simulink model "ELECTRIC_DRIVE"  (R2023a)
settings: Solver=ode1  StartTime=0.0  StopTime=tsim  FixedStep=CONTROL.Tm  RelTol=1e-3
undefined symbols (not defined in the file): CONTROL, MOTOR, myev, SENSOR, speed, tfalta, Tload, Vdc, VSC
libraries: simulink x9
(part 1 of 2)
settings Model: Creator=Usuario  LastModifiedBy=Usuario
settings DataIOCC: TimeSaveName=time  ReturnWorkspaceOutputsName=sim

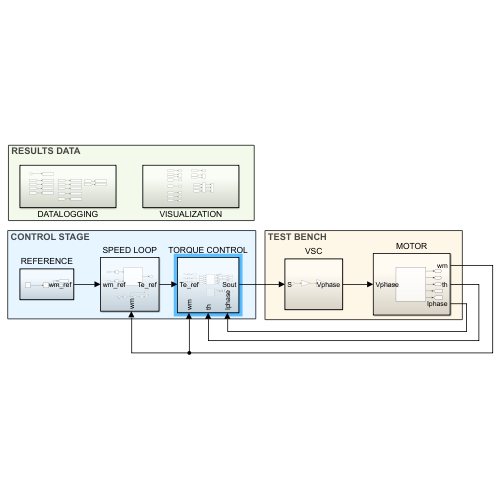
[thumbnail: Simulink's stored preview of the top-level diagram]
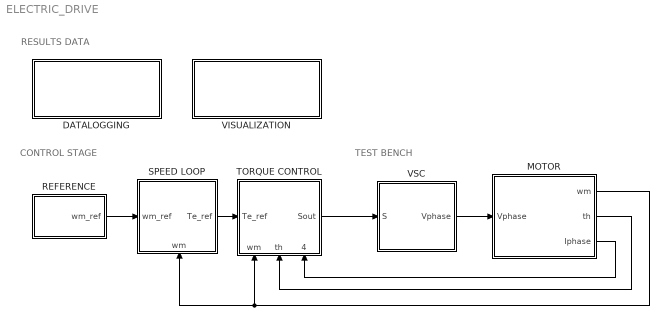
== system ELECTRIC_DRIVE ==
  note: RESULTS DATA
  note: TEST BENCH
  note: CONTROL STAGE
  DATALOGGING : Subsystem
  MOTOR : Subsystem
  REFERENCE : Subsystem
  SPEED LOOP : Subsystem
      settings: PortSchema="{\"entries\":[{\"content\":{\"sides\":[{\"content\":{\"connectorIds\":[\"In1\"]},\"type\":\"ConnectorPlacement.EquallySpacedRectSide\",\"uuid\":\"5121667f-51ba-4a0e-bd85-e87565fa1906\"},{\"content\":{\"connectorIds\":[\"Out1\"],\"side\":\"RIGHT\"},\"type\":\"ConnectorPlacement.EquallySpacedRectSide\",\"uuid\":\"7524861e-419c-49c4-ae4b-3a063630bebd\"},{\"content\":{\"side\":\"TOP\"},\"type\":\"ConnectorPlacement.EquallySpacedRectSide\",\"uuid\":\"8ed52486-91aa-4ff3-9364-bb7dbd5470e8\"},{\"content\":{\"connectorIds\":[\"In2\"],\"side\":\"BOTTOM\"},\"type\":\"ConnectorPlacement.EquallySpacedRectSide\",\"uuid\":\"0ee20b11-26ff-4e27-85a1-93f0e59c0d97\"}]},\"type\":\"ConnectorPlacement.EquallySpacedConnector\",\"uuid\":\"d6389f0f-3d9e-4163-a0bb-1bac6482b2ca\"}],\"packageUris\":[\"http://schema.mathworks.com/mf0/Connector/R2020b\"],\"version\":\"1.0\"}"
  TORQUE CONTROL : Subsystem
      settings: PortSchema="{\"entries\":[{\"content\":{\"sides\":[{\"content\":{\"connectorIds\":[\"In1\"]},\"type\":\"ConnectorPlacement.EquallySpacedRectSide\",\"uuid\":\"5121667f-51ba-4a0e-bd85-e87565fa1906\"},{\"content\":{\"connectorIds\":[\"Out1\"],\"side\":\"RIGHT\"},\"type\":\"ConnectorPlacement.EquallySpacedRectSide\",\"uuid\":\"7524861e-419c-49c4-ae4b-3a063630bebd\"},{\"content\":{\"side\":\"TOP\"},\"type\":\"ConnectorPlacement.EquallySpacedRectSide\",\"uuid\":\"8ed52486-91aa-4ff3-9364-bb7dbd5470e8\"},{\"content\":{\"connectorIds\":[\"In2\",\"In3\",\"In4\"],\"side\":\"BOTTOM\"},\"type\":\"ConnectorPlacement.EquallySpacedRectSide\",\"uuid\":\"eb3bd53b-f837-4c03-9b9f-2d851a494840\"}]},\"type\":\"ConnectorPlacement.EquallySpacedConnector\",\"uuid\":\"d6389f0f-3d9e-4163-a0bb-1bac6482b2ca\"}],\"packageUris\":[\"http://schema.mathworks.com/mf0/Connector/R2020b\"],\"version\":\"1.0\"}"
  VISUALIZATION : Subsystem
  VSC : Subsystem
  wires:
  REFERENCE/1(wm_ref) -> SPEED LOOP/1(wm_ref)
  SPEED LOOP/1(Te_ref) -> TORQUE CONTROL/1(Te_ref)
  TORQUE CONTROL/1(Sout) -> VSC/1(S)
  VSC/1(Vphase) -> MOTOR/1(Vphase)
  MOTOR/3(Iphase) -> TORQUE CONTROL/4(Iphase)
  MOTOR/1(wm) -> SPEED LOOP/2(wm), TORQUE CONTROL/2(wm)
  MOTOR/2(th) -> TORQUE CONTROL/3(th)

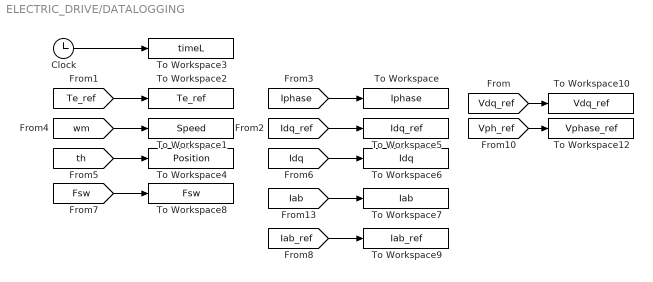
== system ELECTRIC_DRIVE/DATALOGGING ==
  Clock : Clock
  To Workspace : ToWorkspace  VariableName=Iphase  SampleTime=-1
      settings: Decimation=DEC
  To Workspace1 : ToWorkspace  VariableName=Speed  SampleTime=-1
      settings: Decimation=DEC
  To Workspace10 : ToWorkspace  VariableName=Vdq_ref  SampleTime=-1
      settings: Decimation=DEC
  To Workspace12 : ToWorkspace  VariableName=Vphase_ref  SampleTime=-1
      settings: Decimation=DEC
  To Workspace2 : ToWorkspace  VariableName=Te_ref  SampleTime=-1
      settings: Decimation=DEC
  To Workspace3 : ToWorkspace  VariableName=timeL  SampleTime=-1
      settings: Decimation=DEC
  To Workspace4 : ToWorkspace  VariableName=Position  SampleTime=-1
      settings: Decimation=DEC
  To Workspace5 : ToWorkspace  VariableName=Idq_ref  SampleTime=-1
      settings: Decimation=DEC
  To Workspace6 : ToWorkspace  VariableName=Idq  SampleTime=-1
      settings: Decimation=DEC
  To Workspace7 : ToWorkspace  VariableName=Iab  SampleTime=-1
      settings: Decimation=DEC
  To Workspace8 : ToWorkspace  VariableName=Fsw  SampleTime=-1
      settings: Decimation=DEC*100
  To Workspace9 : ToWorkspace  VariableName=Iab_ref  SampleTime=-1
      settings: Decimation=DEC
  wires:
  [Iphase] -> To Workspace/1
  [wm] -> To Workspace1/1
  Clock/1 -> To Workspace3/1
  [Te_ref] -> To Workspace2/1
  [th] -> To Workspace4/1
  [Idq_ref] -> To Workspace5/1
  [Idq] -> To Workspace6/1
  [Iab] -> To Workspace7/1
  [Fsw] -> To Workspace8/1
  [Iab_ref] -> To Workspace9/1
  [Vdq_ref] -> To Workspace10/1
  [Vph_ref] -> To Workspace12/1

== system ELECTRIC_DRIVE/MOTOR ==
  Vphase : Inport
  Variant Subsystem : Subsystem  Variant=on
  wm : Outport
  th : Outport  Port=2
  Iphase : Outport  Port=3
  tag scope: Iab=global, Idq=global
  wires:
  Vphase/1 -> Variant Subsystem/1(Vphase)
  Variant Subsystem/1(wm) -> wm/1
  Variant Subsystem/2(th) -> th/1
  Variant Subsystem/5(Iab) -> [Iab]
  Variant Subsystem/4(Idq) -> [Idq]
  Variant Subsystem/3(Iphase) -> Iphase/1

== system ELECTRIC_DRIVE/REFERENCE ==
  Ramp : simulink/Sources/Ramp  slope=14*speed*2*pi/60  start=0  InitialOutput=0
  Saturation : Saturate  UpperLimit=speed*2*pi/60  LowerLimit=0
  wm_ref : Outport
  tag scope: wm_ref=global
  wires:
  Ramp/1 -> Saturation/1
  Saturation/1 -> [wm_ref], wm_ref/1

== system ELECTRIC_DRIVE/SPEED LOOP ==
  wm_ref : Inport
  wm : Inport  Port=2
  Add : Sum  Commented=on
  Integrator : Integrator  Commented=on
  Ki : Gain  Commented=on  Gain=CONTROL.VEL.Ki
  Kp : Gain  Commented=on  Gain=CONTROL.VEL.Kp
  SPEED PI CONTROLLER : MATLAB Function  Description=OEW MPC VV 5PH  TreatAsAtomicUnit=on
  Sum : Sum  Commented=on  Inputs=|+-
  Transport Delay : TransportDelay  DelayTime=CONTROL.Ts - CONTROL.Tm
  Transport Delay1 : TransportDelay  DelayTime=CONTROL.Ts - CONTROL.Tm
  Te_ref : Outport
  wires:
  Sum/1 -> Kp/1
  Ki/1 -> Integrator/1
  Integrator/1 -> Add/2
  Kp/1 -> Add/1, Ki/1
  wm_ref/1 -> Transport Delay/1
  wm/1 -> Transport Delay1/1
  SPEED PI CONTROLLER/1(T_ref) -> Te_ref/1
  Transport Delay/1 -> SPEED PI CONTROLLER/1(wm_ref)
  Transport Delay1/1 -> SPEED PI CONTROLLER/2(wm)

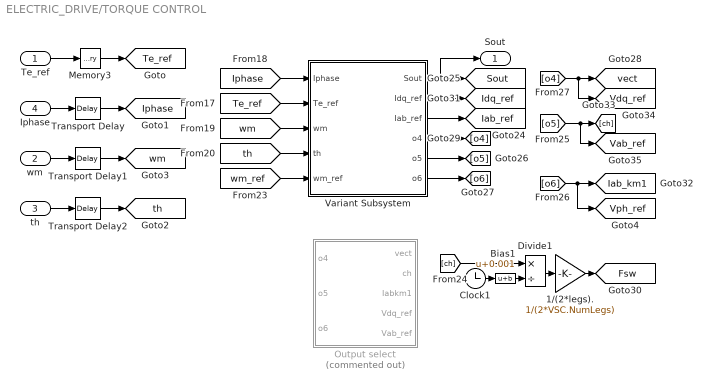
== system ELECTRIC_DRIVE/TORQUE CONTROL ==
  Te_ref : Inport
  wm : Inport  Port=2
  th : Inport  Port=3
  Iphase : Inport  Port=4
  1/(2*legs). : Gain  Gain=1/(2*VSC.NumLegs)
  Bias1 : Bias  Bias=0.001  SaturateOnIntegerOverflow=off
  Clock1 : Clock
  Divide1 : Product  Inputs=*/
  Memory3 : Memory
  Output select : MATLAB Function  Commented=on  TreatAsAtomicUnit=on
  Transport Delay : TransportDelay  DelayTime=CONTROL.Ts - CONTROL.Tm
  Transport Delay1 : TransportDelay  DelayTime=CONTROL.Ts - CONTROL.Tm
  Transport Delay2 : TransportDelay  DelayTime=CONTROL.Ts - CONTROL.Tm
  Variant Subsystem : Subsystem  Variant=on
  Sout : Outport
  tag scope: Fsw=global, Iab_km1=global, Iab_ref=global, Idq_ref=global, Iphase=global, Sout=global, Te_ref=global, Vab_ref=global, Vdq_ref=global, Vph_ref=global, th=global, vect=global, wm=global
  wires:
  Te_ref/1 -> Memory3/1
  Iphase/1 -> Transport Delay/1
  wm/1 -> Transport Delay1/1
  Transport Delay/1 -> [Iphase]
  Memory3/1 -> [Te_ref]
  th/1 -> Transport Delay2/1
  Transport Delay1/1 -> [wm]
  Transport Delay2/1 -> [th]
  [Iphase] -> Variant Subsystem/1(Iphase)
  [Te_ref] -> Variant Subsystem/2(Te_ref)
  [wm] -> Variant Subsystem/3(wm)
  [th] -> Variant Subsystem/4(th)
  [wm_ref] -> Variant Subsystem/5(wm_ref)
  Clock1/1 -> Bias1/1
  Bias1/1 -> Divide1/2
  1/(2*legs)./1 -> [Fsw]
  Divide1/1 -> 1/(2*legs)./1
  Variant Subsystem/1(Sout) -> Sout/1, [Sout]
  Variant Subsystem/4(o4) -> [o4]
  Variant Subsystem/2(Idq_ref) -> [Idq_ref]
  Variant Subsystem/3(Iab_ref) -> [Iab_ref]
  Variant Subsystem/6(o6) -> [o6]
  Variant Subsystem/5(o5) -> [o5]
  [ch] -> Divide1/1
  [o4] -> [Vdq_ref], [vect]
  [o5] -> [Vab_ref], [ch]
  [o6] -> [Vph_ref], [Iab_km1]

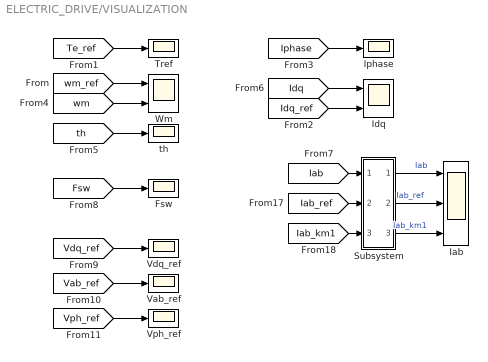
== system ELECTRIC_DRIVE/VISUALIZATION ==
  Fsw : Scope
  Iab : Scope  NumInputPorts=3
  Idq : Scope  NumInputPorts=2
  Iphase : Scope
  Subsystem : Subsystem
  Tref : Scope
  Vab_ref : Scope
  Vdq_ref : Scope
  Vph_ref : Scope
  Wm : Scope  NumInputPorts=2
  th : Scope
  wires:
  [th] -> th/1
  [Te_ref] -> Tref/1
  [wm] -> Wm/2
  [Iphase] -> Iphase/1
  [wm_ref] -> Wm/1
  [Iab] -> Subsystem/1(In1)
  [Iab_ref] -> Subsystem/2(In2)
  [Iab_km1] -> Subsystem/3(In3)
  Subsystem/1(Out1) -> Iab/1  "Iab"
  Subsystem/2(Out2) -> Iab/2  "Iab_ref"
  Subsystem/3(Out3) -> Iab/3  "Iab_km1"
  [Fsw] -> Fsw/1
  [Vdq_ref] -> Vdq_ref/1
  [Vab_ref] -> Vab_ref/1
  [Vph_ref] -> Vph_ref/1
  [Idq] -> Idq/1
  [Idq_ref] -> Idq/2

== system ELECTRIC_DRIVE/VSC ==
  S : Inport
  VSC Model : Gain  Gain=VSC.K  Multiplication=Matrix(K*u)
  Vdc : Gain  Gain=VSC.Vdc
  Vphase : Outport
  wires:
  S/1 -> Vdc/1
  VSC Model/1 -> Vphase/1
  Vdc/1 -> VSC Model/1

== system ELECTRIC_DRIVE/MOTOR/Variant Subsystem ==
  note: 1) Add Subsystem or Model blocks as valid variant choices.
      | 2) You cannot connect blocks at this level. At simulation, connectivity is automatically
      | determined, based on the active variant and port name matching.
  Vphase : Inport
  IM_5Ph : Subsystem  VariantControl=MOTOR.Index == 2
  IM_6Ph : Subsystem  VariantControl=MOTOR.Index == 6
  PMSM_5Ph : Subsystem  VariantControl=MOTOR.Index == 1
  PMSM_9Ph : Subsystem  VariantControl=MOTOR.Index == 3
  wm : Outport
  th : Outport  Port=2
  Iphase : Outport  Port=3
  Idq : Outport  Port=4
  Iab : Outport  Port=5

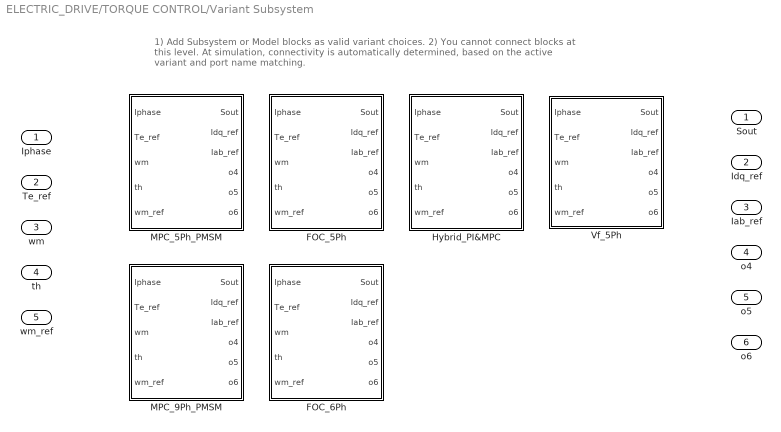
== system ELECTRIC_DRIVE/TORQUE CONTROL/Variant Subsystem ==
  note: 1) Add Subsystem or Model blocks as valid variant choices.
      | 2) You cannot connect blocks at this level. At simulation, connectivity is automatically
      | determined, based on the active variant and port name matching.
  Iphase : Inport
  Te_ref : Inport  Port=2
  wm : Inport  Port=3
  th : Inport  Port=4
  wm_ref : Inport  Port=5
  FOC_5Ph : Subsystem  VariantControl=CONTROL.Index == 52
  FOC_6Ph : Subsystem  VariantControl=CONTROL.Index == 52
  Hybrid_PI&MPC : Subsystem  VariantControl=CONTROL.Index == 53
  MPC_5Ph_PMSM : Subsystem  VariantControl=CONTROL.Index == 51
  MPC_9Ph_PMSM : Subsystem  VariantControl=CONTROL.Index == 91
  Vf_5Ph : Subsystem  VariantControl=CONTROL.Index == 55
  Sout : Outport
  Idq_ref : Outport  Port=2
  Iab_ref : Outport  Port=3
  o4 : Outport  Port=4
  o5 : Outport  Port=5
  o6 : Outport  Port=6

== system ELECTRIC_DRIVE/VISUALIZATION/Subsystem ==
  In1 : Inport
  In2 : Inport  Port=2
  In3 : Inport  Port=3
  Demux1 : Demux  Outputs=[2 3]
  Demux2 : Demux  Outputs=[2 3]
  Out1 : Outport
  Out2 : Outport  Port=2
  Out3 : Outport  Port=3
  wires:
  In1/1 -> Out1/1
  In2/1 -> Demux1/1
  In3/1 -> Demux2/1
  Demux2/1 -> Out3/1
  Demux1/1 -> Out2/1

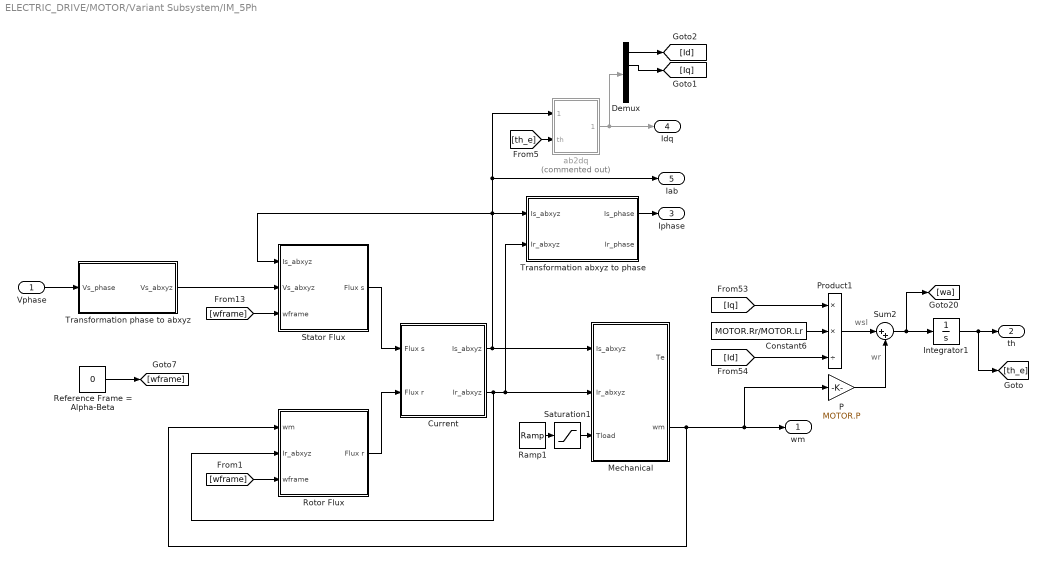
== system ELECTRIC_DRIVE/MOTOR/Variant Subsystem/IM_5Ph ==
  note: wr
  note: wsl
  Vphase : Inport
  Constant6 : Constant  Value=MOTOR.Rr/MOTOR.Lr
  Current : Subsystem
  Demux : Demux
  Integrator1 : Integrator
  Mechanical : Subsystem
  P : Gain  Gain=MOTOR.P
  Product1 : Product  Inputs=**/  RndMeth=Zero
  Ramp1 : simulink/Sources/Ramp  slope=40*Tload  start=0  InitialOutput=0
  Reference Frame = Alpha-Beta : Constant  Value=0
  Rotor Flux : Subsystem
  Saturation1 : Saturate  UpperLimit=Tload  LowerLimit=0
  "Stator Flux " : Subsystem
  Sum2 : Sum  Inputs=|++
  Transformation abxyz to phase : Subsystem
  Transformation phase to abxyz : Subsystem
  ab2dq : MATLAB Function  Commented=on  TreatAsAtomicUnit=on
  wm : Outport  VectorParamsAs1DForOutWhenUnconnected=off
  th : Outport  Port=2  VectorParamsAs1DForOutWhenUnconnected=off
  Iphase : Outport  Port=3  VectorParamsAs1DForOutWhenUnconnected=off
  Idq : Outport  Port=4  VectorParamsAs1DForOutWhenUnconnected=off
  Iab : Outport  Port=5  VectorParamsAs1DForOutWhenUnconnected=off
  wires:
  [wframe] -> "Stator Flux "/3(wframe)
  Transformation phase to abxyz/1(Vs_abxyz) -> "Stator Flux "/2(Vs_abxyz)
  Ramp1/1 -> Saturation1/1
  Vphase/1 -> Transformation phase to abxyz/1(Vs_phase)
  Current/2(Ir_abxyz) -> Rotor Flux/2(Ir_abxyz), Transformation abxyz to phase/2(Ir_abxyz), Mechanical/2(Ir_abxyz)
  Current/1(Is_abxyz) -> ab2dq/1(Vabxy), Iab/1, Transformation abxyz to phase/1(Is_abxyz), "Stator Flux "/1(Is_abxyz), Mechanical/1(Is_abxyz)
  "Stator Flux "/1(Flux s) -> Current/1(Flux s)
  Reference Frame = Alpha-Beta/1 -> [wframe]
  Rotor Flux/1(Flux r) -> Current/2(Flux r)
  [wframe] -> Rotor Flux/3(wframe)
  Saturation1/1 -> Mechanical/3(Tload)
  Transformation abxyz to phase/1(Is_phase) -> Iphase/1
  Integrator1/1 -> [th_e], th/1
  [th_e] -> ab2dq/2(th)
  ab2dq/1(Vdqxy) -> Demux/1, Idq/1
  P/1 -> Sum2/2
  Product1/1 -> Sum2/1
  [Id] -> Product1/3
  Mechanical/2(wm) -> P/1, wm/1, Rotor Flux/1(wm)
  Sum2/1 -> Integrator1/1, [wa]
  Constant6/1 -> Product1/2
  [Iq] -> Product1/1
  Demux/2 -> [Iq]
  Demux/1 -> [Id]

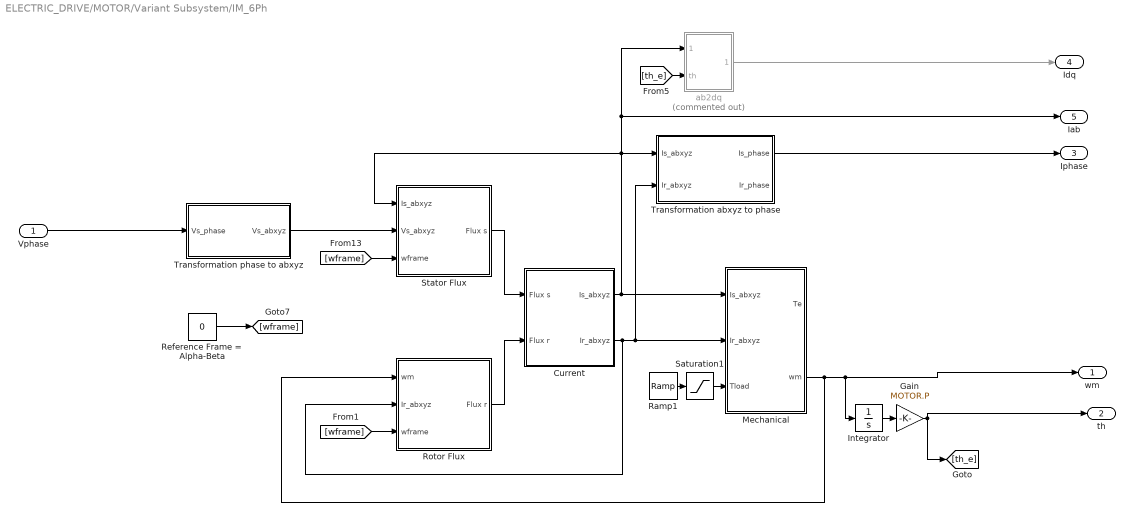
== system ELECTRIC_DRIVE/MOTOR/Variant Subsystem/IM_6Ph ==
  Vphase : Inport
  Current : Subsystem
  Gain : Gain  Gain=MOTOR.P
  Integrator : Integrator
  Mechanical : Subsystem
  Ramp1 : simulink/Sources/Ramp  slope=40*Tload  start=0  InitialOutput=0
  Reference Frame = Alpha-Beta : Constant  Value=0
  Rotor Flux : Subsystem
  Saturation1 : Saturate  UpperLimit=Tload  LowerLimit=0
  "Stator Flux " : Subsystem
  Transformation abxyz to phase : Subsystem
  Transformation phase to abxyz : Subsystem
  ab2dq : MATLAB Function  Commented=on  TreatAsAtomicUnit=on
  wm : Outport  VectorParamsAs1DForOutWhenUnconnected=off
  th : Outport  Port=2  VectorParamsAs1DForOutWhenUnconnected=off
  Iphase : Outport  Port=3  VectorParamsAs1DForOutWhenUnconnected=off
  Idq : Outport  Port=4  VectorParamsAs1DForOutWhenUnconnected=off
  Iab : Outport  Port=5  VectorParamsAs1DForOutWhenUnconnected=off
  wires:
  ab2dq/1(Vdqxy) -> Idq/1
  [th_e] -> ab2dq/2(th)
  Gain/1 -> th/1, [th_e]
  Integrator/1 -> Gain/1
  Transformation abxyz to phase/1(Is_phase) -> Iphase/1
  Saturation1/1 -> Mechanical/3(Tload)
  [wframe] -> Rotor Flux/3(wframe)
  Rotor Flux/1(Flux r) -> Current/2(Flux r)
  Mechanical/2(wm) -> Rotor Flux/1(wm), wm/1, Integrator/1
  Reference Frame = Alpha-Beta/1 -> [wframe]
  "Stator Flux "/1(Flux s) -> Current/1(Flux s)
  Current/1(Is_abxyz) -> Mechanical/1(Is_abxyz), "Stator Flux "/1(Is_abxyz), Transformation abxyz to phase/1(Is_abxyz), Iab/1, ab2dq/1(Vabxy)
  Current/2(Ir_abxyz) -> Mechanical/2(Ir_abxyz), Transformation abxyz to phase/2(Ir_abxyz), Rotor Flux/2(Ir_abxyz)
  Vphase/1 -> Transformation phase to abxyz/1(Vs_phase)
  Ramp1/1 -> Saturation1/1
  Transformation phase to abxyz/1(Vs_abxyz) -> "Stator Flux "/2(Vs_abxyz)
  [wframe] -> "Stator Flux "/3(wframe)

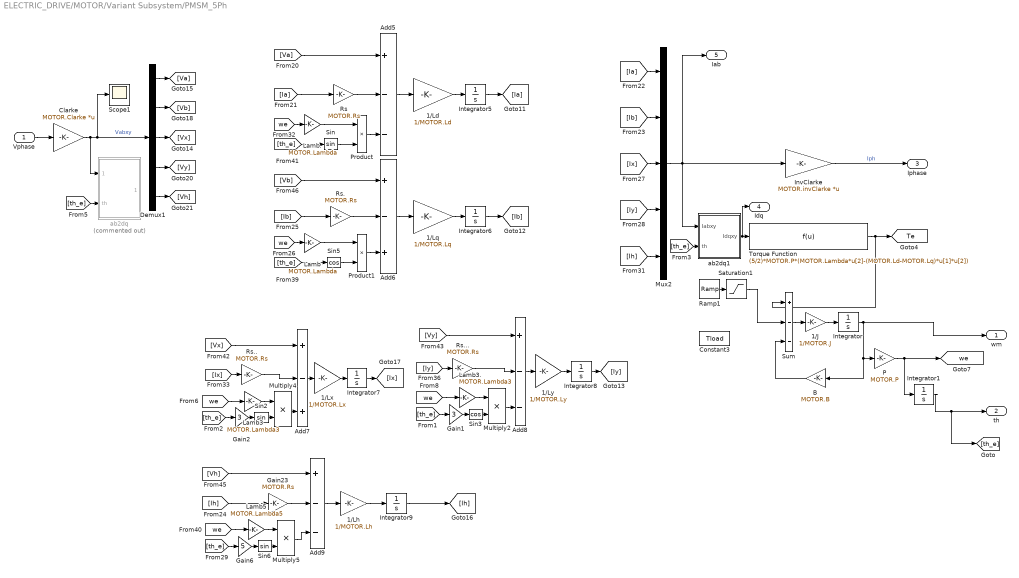
== system ELECTRIC_DRIVE/MOTOR/Variant Subsystem/PMSM_5Ph ==
  Vphase : Inport
  1/J : Gain  Gain=1/MOTOR.J
  1/Ld : Gain  Gain=1/MOTOR.Ld
  1/Lh : Gain  Gain=1/MOTOR.Lh
  1/Lq : Gain  Gain=1/MOTOR.Lq
  1/Lx : Gain  Gain=1/MOTOR.Lx
  1/Ly : Gain  Gain=1/MOTOR.Ly
  Add5 : Sum  Inputs=+--
  Add6 : Sum  Inputs=+-+
  Add7 : Sum  Inputs=+-+
  Add8 : Sum  Inputs=+--
  Add9 : Sum  Inputs=+--
  B : Gain  Gain=MOTOR.B
  Clarke : Gain  Gain=MOTOR.Clarke  Multiplication=Matrix(K*u)
  Constant3 : Constant  Value=Tload
  Demux1 : Demux  Outputs=5
  Gain1 : Gain  Gain=3
  Gain2 : Gain  Gain=3
  Gain23 : Gain  Gain=MOTOR.Rs
  Gain6 : Gain  Gain=5
  Integrator{,1,5..9} (7 alike) : Integrator
  InvClarke : Gain  Gain=MOTOR.invClarke  Multiplication=Matrix(K*u)
  Lamb : Gain  Gain=MOTOR.Lambda
  Lamb. : Gain  Gain=MOTOR.Lambda
  Lamb3 : Gain  Gain=MOTOR.Lambda3
  Lamb3. : Gain  Gain=MOTOR.Lambda3
  Lamb5 : Gain  Gain=MOTOR.Lambda5
  Multiply2 : Product
  Multiply4 : Product
  Multiply5 : Product
  Mux2 : Mux  Inputs=5
  P : Gain  Gain=MOTOR.P
  Product : Product
  Product1 : Product
  Ramp1 : simulink/Sources/Ramp  slope=40*Tload  start=0  InitialOutput=0
  Rs : Gain  Gain=MOTOR.Rs
  Rs. : Gain  Gain=MOTOR.Rs
  Rs.. : Gain  Gain=MOTOR.Rs
  Rs... : Gain  Gain=MOTOR.Rs
  Saturation1 : Saturate  UpperLimit=Tload  LowerLimit=0
  Scope1 : Scope
  Sin : Trigonometry
  Sin2 : Trigonometry
  Sin3 : Trigonometry  Operator=cos
  Sin5 : Trigonometry  Operator=cos
  Sin6 : Trigonometry
  Sum : Sum  Inputs=+--
  Torque Function : Fcn  Expr=(5/2)*MOTOR.P*(MOTOR.Lambda*u[2]-(MOTOR.Ld-MOTOR.Lq)*u[1]*u[2])
  ab2dq : MATLAB Function  Commented=on  TreatAsAtomicUnit=on
  ab2dq1 : MATLAB Function  TreatAsAtomicUnit=on
  wm : Outport
  th : Outport  Port=2
  Iphase : Outport  Port=3
  Idq : Outport  Port=4
  Iab : Outport  Port=5
  tag scope: Te=global, we=global
  wires:
  Gain6/1 -> Sin6/1
  [we] -> Lamb5/1
  Ramp1/1 -> Saturation1/1
  Sin6/1 -> Multiply5/2
  [Va] -> Add5/1
  Lamb5/1 -> Multiply5/1
  Gain1/1 -> Sin3/1
  Lamb3./1 -> Multiply2/1
  1/Lq/1 -> Integrator6/1
  Add8/1 -> 1/Ly/1
  [th_e] -> Gain1/1
  [th_e] -> Gain6/1
  [we] -> Lamb3./1
  Add6/1 -> 1/Lq/1
  [Ix] -> Mux2/3
  Sin/1 -> Product/2
  [th_e] -> Sin/1
  Vphase/1 -> Clarke/1
  1/Ly/1 -> Integrator8/1
  [th_e] -> Sin5/1
  Integrator8/1 -> [Iy]
  Multiply2/1 -> Add8/3
  [we] -> Lamb/1
  Demux1/3 -> [Vx]
  Sin3/1 -> Multiply2/2
  Lamb/1 -> Product1/1
  Sin5/1 -> Product1/2
  ab2dq1/1(Idqxy) -> Torque Function/1, Idq/1
  Rs/1 -> Add5/2
  Rs.../1 -> Add8/2
  Integrator5/1 -> [Ia]
  [Ih] -> Gain23/1
  [we] -> Lamb./1
  [th_e] -> ab2dq/2(th)
  [th_e] -> ab2dq1/2(th)
  [Ib] -> Rs./1
  Rs../1 -> Add7/2
  B/1 -> Sum/3
  InvClarke/1 -> Iphase/1  "Iph"
  Product/1 -> Add5/3
  [Vb] -> Add6/1
  1/Lh/1 -> Integrator9/1
  [Ia] -> Rs/1
  Add9/1 -> 1/Lh/1
  Demux1/2 -> [Vb]
  [Vh] -> Add9/1
  Integrator/1 -> P/1, B/1, wm/1
  Torque Function/1 -> [Te], Sum/1
  Saturation1/1 -> Sum/2
  Integrator1/1 -> [th_e], th/1
  1/Lx/1 -> Integrator7/1
  Sum/1 -> 1/J/1
  Clarke/1 -> Scope1/1, Demux1/1, ab2dq/1(Vabxy)  "Vabxy"
  [Ia] -> Mux2/1
  Lamb3/1 -> Multiply4/1
  [Ib] -> Mux2/2
  Add5/1 -> 1/Ld/1
  [Ih] -> Mux2/5
  Product1/1 -> Add6/3
  Add7/1 -> 1/Lx/1
  Rs./1 -> Add6/2
  Integrator9/1 -> [Ih]
  [th_e] -> Gain2/1
  [Iy] -> Mux2/4
  1/Ld/1 -> Integrator5/1
  1/J/1 -> Integrator/1
  Integrator7/1 -> [Ix]
  Demux1/5 -> [Vh]
  Gain23/1 -> Add9/2
  Integrator6/1 -> [Ib]
  Demux1/1 -> [Va]
  P/1 -> Integrator1/1, [we]
  [Iy] -> Rs.../1
  Mux2/1 -> InvClarke/1, ab2dq1/1(Iabxy), Iab/1
  Lamb./1 -> Product/1
  [Vy] -> Add8/1
  Gain2/1 -> Sin2/1
  Demux1/4 -> [Vy]
  Multiply5/1 -> Add9/3
  [we] -> Lamb3/1
  [Ix] -> Rs../1
  [Vx] -> Add7/1
  Multiply4/1 -> Add7/3
  Sin2/1 -> Multiply4/2

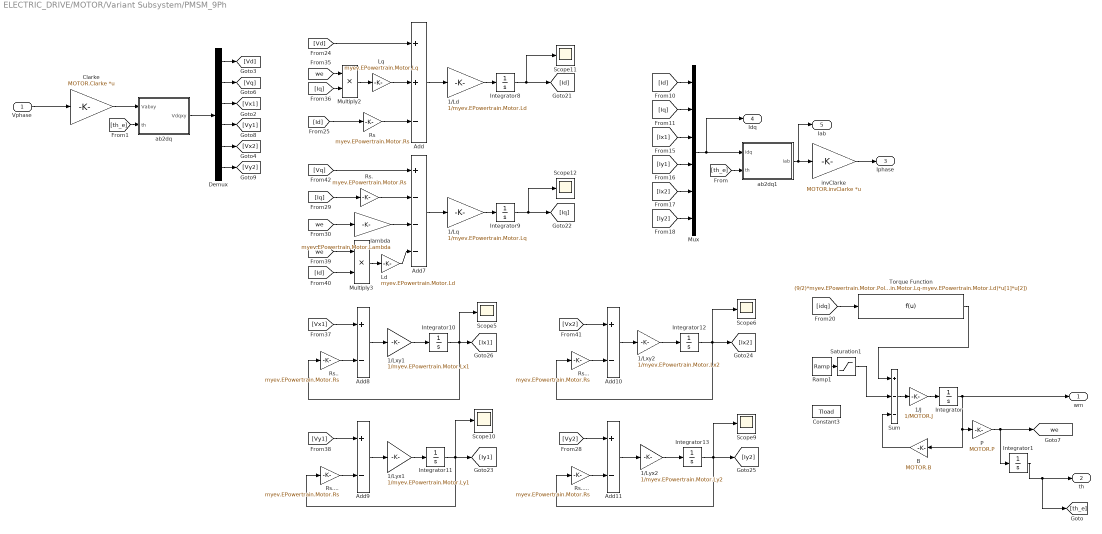
== system ELECTRIC_DRIVE/MOTOR/Variant Subsystem/PMSM_9Ph ==
  Vphase : Inport
  1/J : Gain  Gain=1/MOTOR.J
  1/Ld : Gain  Gain=1/myev.EPowertrain.Motor.Ld
  1/Lq : Gain  Gain=1/myev.EPowertrain.Motor.Lq
  1/Lxy1 : Gain  Gain=1/myev.EPowertrain.Motor.Lx1
  1/Lxy2 : Gain  Gain=1/myev.EPowertrain.Motor.Lx2
  1/Lyx1 : Gain  Gain=1/myev.EPowertrain.Motor.Ly1
  1/Lyx2 : Gain  Gain=1/myev.EPowertrain.Motor.Ly2
  Add : Sum  Inputs=++-
  Add{8..11} (4 alike) : Sum  Inputs=+-
  Add7 : Sum  Inputs=+---
  B : Gain  Gain=MOTOR.B
  Clarke : Gain  Gain=MOTOR.Clarke  Multiplication=Matrix(K*u)
  Constant3 : Constant  Value=Tload
  Demux : Demux  Outputs=6
  Integrator{,1,8..13} (8 alike) : Integrator
  Ld : Gain  Gain=myev.EPowertrain.Motor.Ld
  Lq : Gain  Gain=myev.EPowertrain.Motor.Lq
  Multiply2 : Product
  Multiply3 : Product
  Mux : Mux  Inputs=6
  P : Gain  Gain=MOTOR.P
  Ramp1 : simulink/Sources/Ramp  slope=40*Tload  start=0  InitialOutput=0
  Rs : Gain  Gain=myev.EPowertrain.Motor.Rs
  Rs. : Gain  Gain=myev.EPowertrain.Motor.Rs
  Rs.. : Gain  Gain=myev.EPowertrain.Motor.Rs
  Rs... : Gain  Gain=myev.EPowertrain.Motor.Rs
  Rs.... : Gain  Gain=myev.EPowertrain.Motor.Rs
  Rs..... : Gain  Gain=myev.EPowertrain.Motor.Rs
  Saturation1 : Saturate  UpperLimit=Tload  LowerLimit=0
  Scope{5..6,9..12} (6 alike) : Scope
  Sum : Sum  Inputs=+--
  Torque Function : Fcn  Expr=(9/2)*myev.EPowertrain.Motor.Poles*(myev.EPowertrain.Motor.Lambda*u[2]-(myev.EPowertrain.Motor.Lq-myev.EPowertrain.Motor.Ld)*u[1]*u[2])
  ab2dq : MATLAB Function  TreatAsAtomicUnit=on
  ab2dq1 : MATLAB Function  TreatAsAtomicUnit=on
  invClarke : Gain  Gain=MOTOR.invClarke  Multiplication=Matrix(K*u)
  lambda : Gain  Gain=myev.EPowertrain.Motor.Lambda
  wm : Outport
  th : Outport  Port=2
  Iphase : Outport  Port=3
  Idq : Outport  Port=4
  Iab : Outport  Port=5
  tag scope: we=global
  wires:
  Vphase/1 -> Clarke/1
  1/Ld/1 -> Integrator8/1
  Demux/5 -> [Vx2]
  Integrator10/1 -> Rs../1, [Ix1], Scope5/1
  Add10/1 -> 1/Lxy2/1
  [idq] -> Torque Function/1
  Integrator9/1 -> Scope12/1, [Iq]
  [Id] -> Rs/1
  Integrator8/1 -> Scope11/1, [Id]
  [Vq] -> Add7/1
  Rs./1 -> Add7/2
  [we] -> Multiply2/1
  Multiply3/1 -> Ld/1
  [Iq] -> Multiply2/2
  Demux/4 -> [Vy1]
  Demux/3 -> [Vx1]
  ab2dq/1(Vdqxy) -> Demux/1
  [Ix2] -> Mux/5
  Demux/6 -> [Vy2]
  Clarke/1 -> ab2dq/1(Vabxy)
  Mux/1 -> ab2dq1/1(idq), Idq/1
  Rs.../1 -> Add10/2
  Demux/1 -> [Vd]
  1/Lq/1 -> Integrator9/1
  Add9/1 -> 1/Lyx1/1
  [we] -> lambda/1
  lambda/1 -> Add7/3
  Demux/2 -> [Vq]
  [Vy2] -> Add11/1
  Multiply2/1 -> Lq/1
  Rs/1 -> Add/3
  Rs..../1 -> Add9/2
  [Id] -> Multiply3/2
  [Vy1] -> Add9/1
  Integrator11/1 -> Scope10/1, Rs..../1, [Iy1]
  Rs...../1 -> Add11/2
  Integrator13/1 -> Scope9/1, Rs...../1, [Iy2]
  [Iq] -> Rs./1
  1/Lxy1/1 -> Integrator10/1
  [Vd] -> Add/1
  1/Lxy2/1 -> Integrator12/1
  [Id] -> Mux/1
  Add8/1 -> 1/Lxy1/1
  [Iy1] -> Mux/4
  1/Lyx2/1 -> Integrator13/1
  [Vx1] -> Add8/1
  [Iq] -> Mux/2
  Add7/1 -> 1/Lq/1
  [we] -> Multiply3/1
  Integrator12/1 -> Scope6/1, [Ix2], Rs.../1
  [Ix1] -> Mux/3
  1/Lyx1/1 -> Integrator11/1
  Rs../1 -> Add8/2
  [Iy2] -> Mux/6
  [Vx2] -> Add10/1
  Ld/1 -> Add7/4
  Add11/1 -> 1/Lyx2/1
  Lq/1 -> Add/2
  Add/1 -> 1/Ld/1
  ab2dq1/1(iab) -> Iab/1, invClarke/1
  invClarke/1 -> Iphase/1
  Ramp1/1 -> Saturation1/1
  Torque Function/1 -> Sum/1
  P/1 -> Integrator1/1, [we]
  B/1 -> Sum/3
  Integrator1/1 -> th/1, [th_e]
  Saturation1/1 -> Sum/2
  1/J/1 -> Integrator/1
  Integrator/1 -> wm/1, P/1, B/1
  Sum/1 -> 1/J/1
  [th_e] -> ab2dq1/2(th)
  [th_e] -> ab2dq/2(th)

== system ELECTRIC_DRIVE/TORQUE CONTROL/Variant Subsystem/FOC_5Ph ==
  Iphase : Inport
  Te_ref : Inport  Port=2
  wm : Inport  Port=3
  th : Inport  Port=4
  wm_ref : Inport  Port=5
  FOC 5Phase PMSM : MATLAB Function  Description=OEW MPC VV 5PH  TreatAsAtomicUnit=on
  MODULATION STAGE : Subsystem
  Sout : Outport
  Idq_ref : Outport  Port=2
  Iab_ref : Outport  Port=3
  o4 : Outport  Port=4
  o5 : Outport  Port=5
  o6 : Outport  Port=6
  wires:
  FOC 5Phase PMSM/3(IabRef) -> Iab_ref/1
  FOC 5Phase PMSM/2(IdqRef) -> Idq_ref/1
  FOC 5Phase PMSM/1(Vph_ref) -> o6/1, MODULATION STAGE/1(Vph)
  th/1 -> FOC 5Phase PMSM/4(th)
  wm/1 -> FOC 5Phase PMSM/3(wm)
  Te_ref/1 -> FOC 5Phase PMSM/2(Tref)
  Iphase/1 -> FOC 5Phase PMSM/1(Iabc_med)
  MODULATION STAGE/1(Sout) -> Sout/1
  FOC 5Phase PMSM/4(VdqRef) -> o4/1
  FOC 5Phase PMSM/5(VabRef) -> o5/1

== system ELECTRIC_DRIVE/TORQUE CONTROL/Variant Subsystem/FOC_6Ph ==
  Iphase : Inport
  Te_ref : Inport  Port=2
  wm : Inport  Port=3
  th : Inport  Port=4
  wm_ref : Inport  Port=5
  FOC 6Phase PMSM : MATLAB Function  Description=OEW MPC VV 5PH  TreatAsAtomicUnit=on
  MODULATION STAGE : Subsystem
  Sout : Outport
  Idq_ref : Outport  Port=2
  Iab_ref : Outport  Port=3
  o4 : Outport  Port=4
  o5 : Outport  Port=5
  o6 : Outport  Port=6
  wires:
  FOC 6Phase PMSM/5(VabRef) -> o5/1
  FOC 6Phase PMSM/4(VdqRef) -> o4/1
  MODULATION STAGE/1(Sout) -> Sout/1
  Iphase/1 -> FOC 6Phase PMSM/1(Iabc_med)
  Te_ref/1 -> FOC 6Phase PMSM/2(Tref)
  wm/1 -> FOC 6Phase PMSM/3(wm)
  th/1 -> FOC 6Phase PMSM/4(th)
  FOC 6Phase PMSM/1(Vph_ref) -> MODULATION STAGE/1(Vph), o6/1
  FOC 6Phase PMSM/2(IdqRef) -> Idq_ref/1
  FOC 6Phase PMSM/3(IabRef) -> Iab_ref/1

== system ELECTRIC_DRIVE/TORQUE CONTROL/Variant Subsystem/Hybrid_PI&MPC ==
  Iphase : Inport
  Te_ref : Inport  Port=2
  wm : Inport  Port=3
  th : Inport  Port=4
  wm_ref : Inport  Port=5
  Hybrid PIdq and MPCh 5Ph : MATLAB Function  Description=OEW MPC VV 5PH  TreatAsAtomicUnit=on
  MODULATION STAGE : Subsystem
  Sout : Outport
  Idq_ref : Outport  Port=2
  Iab_ref : Outport  Port=3
  o4 : Outport  Port=4
  o5 : Outport  Port=5
  o6 : Outport  Port=6
  wires:
  Hybrid PIdq and MPCh 5Ph/5(VabRef) -> o5/1
  Hybrid PIdq and MPCh 5Ph/4(VdqRef) -> o4/1
  MODULATION STAGE/1(Sout) -> Sout/1
  Iphase/1 -> Hybrid PIdq and MPCh 5Ph/1(Iabc_med)
  Te_ref/1 -> Hybrid PIdq and MPCh 5Ph/2(Tref)
  wm/1 -> Hybrid PIdq and MPCh 5Ph/3(wm)
  th/1 -> Hybrid PIdq and MPCh 5Ph/4(th)
  Hybrid PIdq and MPCh 5Ph/1(Vph_ref) -> MODULATION STAGE/1(Vph), o6/1
  Hybrid PIdq and MPCh 5Ph/2(IdqRef) -> Idq_ref/1
  Hybrid PIdq and MPCh 5Ph/3(IabRef) -> Iab_ref/1

== system ELECTRIC_DRIVE/TORQUE CONTROL/Variant Subsystem/MPC_5Ph_PMSM ==
  Iphase : Inport
  Te_ref : Inport  Port=2
  wm : Inport  Port=3
  th : Inport  Port=4
  wm_ref : Inport  Port=5
  MPC 5Phase PMSM : MATLAB Function  Description=OEW MPC VV 5PH  TreatAsAtomicUnit=on
  Sout : Outport
  Idq_ref : Outport  Port=2
  Iab_ref : Outport  Port=3
  o4 : Outport  Port=4
  o5 : Outport  Port=5
  o6 : Outport  Port=6
  wires:
  Iphase/1 -> MPC 5Phase PMSM/1(Iabc_med)
  Te_ref/1 -> MPC 5Phase PMSM/2(Tref)
  wm/1 -> MPC 5Phase PMSM/3(wm)
  th/1 -> MPC 5Phase PMSM/4(th)
  MPC 5Phase PMSM/1(Sout) -> Sout/1
  MPC 5Phase PMSM/4(IdqRef) -> Idq_ref/1
  MPC 5Phase PMSM/5(IabRef) -> Iab_ref/1
  MPC 5Phase PMSM/2(vectores) -> o4/1
  MPC 5Phase PMSM/7(ch) -> o5/1
  MPC 5Phase PMSM/6(Iab_km1) -> o6/1

== system ELECTRIC_DRIVE/TORQUE CONTROL/Variant Subsystem/MPC_9Ph_PMSM ==
  Iphase : Inport
  Te_ref : Inport  Port=2
  wm : Inport  Port=3
  th : Inport  Port=4
  wm_ref : Inport  Port=5
  MPC 9Phase PMSM : MATLAB Function  Description=OEW MPC VV 5PH  TreatAsAtomicUnit=on
  Sout : Outport
  Idq_ref : Outport  Port=2
  Iab_ref : Outport  Port=3
  o4 : Outport  Port=4
  o5 : Outport  Port=5
  o6 : Outport  Port=6
  wires:
  MPC 9Phase PMSM/6(Iab_km1) -> o6/1
  MPC 9Phase PMSM/7(ch) -> o5/1
  MPC 9Phase PMSM/5(IabRef) -> Iab_ref/1
  MPC 9Phase PMSM/4(IdqRef) -> Idq_ref/1
  MPC 9Phase PMSM/2(vectores) -> o4/1
  MPC 9Phase PMSM/1(Sout) -> Sout/1
  th/1 -> MPC 9Phase PMSM/4(th)
  wm/1 -> MPC 9Phase PMSM/3(wm)
  Te_ref/1 -> MPC 9Phase PMSM/2(Tref)
  Iphase/1 -> MPC 9Phase PMSM/1(Iabc_med)

== system ELECTRIC_DRIVE/TORQUE CONTROL/Variant Subsystem/Vf_5Ph ==
  Iphase : Inport
  Te_ref : Inport  Port=2
  wm : Inport  Port=3
  th : Inport  Port=4
  wm_ref : Inport  Port=5
  MODULATOR : Subsystem
  Vf 5Phase PMSM : MATLAB Function  Description=OEW MPC VV 5PH  TreatAsAtomicUnit=on
  Sout : Outport
  Idq_ref : Outport  Port=2
  Iab_ref : Outport  Port=3
  o4 : Outport  Port=4
  o5 : Outport  Port=5
  o6 : Outport  Port=6
  wires:
  Vf 5Phase PMSM/1(Vphase) -> MODULATOR/1(Vphase)
  MODULATOR/1(Sout) -> Sout/1
  wm_ref/1 -> Vf 5Phase PMSM/1(wm)

== system ELECTRIC_DRIVE/MOTOR/Variant Subsystem/IM_5Ph/Current ==
  Flux s : Inport
  Flux r : Inport  Port=2
  1/Kw : Gain  Gain=1/MOTOR.Kw
  Demux : Demux  Outputs=2
  Demux1 : Demux  Outputs=5
  Gain : Gain  Gain=0
  Mux : Mux  Inputs=2
  Mux1 : Mux  Inputs=5
  falta : Subsystem  Commented=on
  invA*u : Gain  Gain=MOTOR.invA  Multiplication=Matrix(K*u)
  Is_abxyz : Outport  VectorParamsAs1DForOutWhenUnconnected=off
  Ir_abxyz : Outport  Port=2  VectorParamsAs1DForOutWhenUnconnected=off
  wires:
  Flux s/1 -> Mux/1
  Flux r/1 -> Mux/2
  Mux/1 -> invA*u/1
  invA*u/1 -> Demux/1
  Demux/2 -> 1/Kw/1
  1/Kw/1 -> Ir_abxyz/1
  Demux1/1 -> [i_alpha], Mux1/1
  Demux1/2 -> Mux1/2
  Demux1/4 -> Mux1/4
  Demux1/5 -> Gain/1
  Mux1/1 -> Is_abxyz/1
  Demux/1 -> Demux1/1
  [i_alpha] -> falta/1(I_alpha)
  Demux1/3 -> Mux1/3, falta/2(Ix)
  Gain/1 -> Mux1/5

== system ELECTRIC_DRIVE/MOTOR/Variant Subsystem/IM_5Ph/Mechanical ==
  Is_abxyz : Inport
  Ir_abxyz : Inport  Port=2
  Tload : Inport  Port=3
  Bm*wm : Gain  Gain=MOTOR.Bm
  Inertia : Gain  Gain=1/MOTOR.J
  Integrator : Integrator
  Mux : Mux  Inputs=2
  Sum : Sum  Inputs=+--
  Torque Function : Fcn  Expr=3*MOTOR.P*MOTOR.Lm*(u[2]*u[6]-u[1]*u[7])
  Te : Outport  VectorParamsAs1DForOutWhenUnconnected=off
  wm : Outport  Port=2  VectorParamsAs1DForOutWhenUnconnected=off
  wires:
  Tload/1 -> Sum/2
  Sum/1 -> Inertia/1
  Inertia/1 -> Integrator/1
  Bm*wm/1 -> Sum/3
  Integrator/1 -> wm/1, Bm*wm/1
  Is_abxyz/1 -> Mux/1
  Ir_abxyz/1 -> Mux/2
  Mux/1 -> Torque Function/1
  Torque Function/1 -> Sum/1, Te/1

== system ELECTRIC_DRIVE/MOTOR/Variant Subsystem/IM_5Ph/Rotor Flux ==
  wm : Inport
  Ir_abxyz : Inport  Port=2
  wframe : Inport  Port=3
  Gain1 : Gain  Gain=[0 1 0 0 0 ; -1 0 0 0 0 ; 0 0 0 0 0 ; 0 0 0 0 0 ;0 0 0 0 0]  Multiplication=Matrix(K*u)
  Integrator : Integrator
  Pole Pairs : Gain  Gain=MOTOR.P
  Product : Product  RndMeth=Zero
  Rr : Gain  Gain=MOTOR.Rr
  Sum : Sum  Inputs=-+
  Sum1 : Sum  Inputs=+-
  Flux r : Outport  VectorParamsAs1DForOutWhenUnconnected=off
  wires:
  Ir_abxyz/1 -> Rr/1
  Product/1 -> Sum1/1
  Rr/1 -> Sum1/2
  wframe/1 -> Sum/2
  Sum1/1 -> Integrator/1
  Integrator/1 -> Flux r/1, Gain1/1
  Gain1/1 -> Product/1
  wm/1 -> Pole Pairs/1
  Pole Pairs/1 -> Sum/1
  Sum/1 -> Product/2

== system ELECTRIC_DRIVE/MOTOR/Variant Subsystem/IM_5Ph/Stator Flux  ==
  Is_abxyz : Inport
  Vs_abxyz : Inport  Port=2
  wframe : Inport  Port=3
  Gain : Gain  Gain=[0 1 0 0 0 ;-1 0 0 0 0 ;0 0 0 0 0 ;0 0 0 0 0 ;0 0 0 0 0]  Multiplication=Matrix(K*u)
  Integrator : Integrator
  Product : Product  RndMeth=Zero
  Rs : Gain  Gain=MOTOR.Rs
  Sum : Sum  Inputs=+-+
  Flux s : Outport  VectorParamsAs1DForOutWhenUnconnected=off
  wires:
  Rs/1 -> Sum/2
  Sum/1 -> Integrator/1
  Integrator/1 -> Gain/1, Flux s/1
  Is_abxyz/1 -> Rs/1
  Vs_abxyz/1 -> Sum/1
  Product/1 -> Sum/3
  wframe/1 -> Product/1
  Gain/1 -> Product/2

== system ELECTRIC_DRIVE/MOTOR/Variant Subsystem/IM_5Ph/Transformation abxyz to phase ==
  Is_abxyz : Inport
  Ir_abxyz : Inport  Port=2
  Gain : Gain  Gain=MOTOR.invClarke  Multiplication=Matrix(K*u)
  Gain1 : Gain  Gain=MOTOR.invClarke  Multiplication=Matrix(K*u)
  Is_phase : Outport  VectorParamsAs1DForOutWhenUnconnected=off
  Ir_phase : Outport  Port=2  VectorParamsAs1DForOutWhenUnconnected=off
  wires:
  Is_abxyz/1 -> Gain/1
  Gain/1 -> Is_phase/1
  Ir_abxyz/1 -> Gain1/1
  Gain1/1 -> Ir_phase/1

== system ELECTRIC_DRIVE/MOTOR/Variant Subsystem/IM_5Ph/Transformation phase to abxyz ==
  Vs_phase : Inport
  Transformation alpha-beta-x-y-z : Gain  Gain=MOTOR.Clarke  Multiplication=Matrix(K*u)
  Vs_abxyz : Outport  VectorParamsAs1DForOutWhenUnconnected=off
  wires:
  Transformation alpha-beta-x-y-z/1 -> Vs_abxyz/1
  Vs_phase/1 -> Transformation alpha-beta-x-y-z/1

== system ELECTRIC_DRIVE/MOTOR/Variant Subsystem/IM_6Ph/Current ==
  Flux s : Inport
  Flux r : Inport  Port=2
  1/Kw : Gain  Gain=1/MOTOR.Kw
  Demux : Demux  Outputs=2
  Mux : Mux  Inputs=2
  invA*u : Gain  Gain=MOTOR.invA  Multiplication=Matrix(K*u)
  Is_abxyz : Outport  VectorParamsAs1DForOutWhenUnconnected=off
  Ir_abxyz : Outport  Port=2  VectorParamsAs1DForOutWhenUnconnected=off
  wires:
  1/Kw/1 -> Ir_abxyz/1
  Demux/2 -> 1/Kw/1
  invA*u/1 -> Demux/1
  Mux/1 -> invA*u/1
  Flux r/1 -> Mux/2
  Flux s/1 -> Mux/1
  Demux/1 -> Is_abxyz/1

== system ELECTRIC_DRIVE/MOTOR/Variant Subsystem/IM_6Ph/Mechanical ==
  Is_abxyz : Inport
  Ir_abxyz : Inport  Port=2
  Tload : Inport  Port=3
  Bm*wm : Gain  Gain=MOTOR.Bm
  Inertia : Gain  Gain=1/MOTOR.J
  Integrator : Integrator
  Mux : Mux  Inputs=2
  Sum : Sum  Inputs=+--
  Torque Function : Fcn  Expr=3*MOTOR.P*MOTOR.Lm*(u[2]*u[6]-u[1]*u[7])
  Te : Outport  VectorParamsAs1DForOutWhenUnconnected=off
  wm : Outport  Port=2  VectorParamsAs1DForOutWhenUnconnected=off
  wires:
  Torque Function/1 -> Te/1, Sum/1
  Mux/1 -> Torque Function/1
  Ir_abxyz/1 -> Mux/2
  Is_abxyz/1 -> Mux/1
  Integrator/1 -> Bm*wm/1, wm/1
  Bm*wm/1 -> Sum/3
  Inertia/1 -> Integrator/1
  Sum/1 -> Inertia/1
  Tload/1 -> Sum/2

== system ELECTRIC_DRIVE/MOTOR/Variant Subsystem/IM_6Ph/Rotor Flux ==
  wm : Inport
  Ir_abxyz : Inport  Port=2
  wframe : Inport  Port=3
  Gain1 : Gain  Gain=[0 1 0 0 0 ; -1 0 0 0 0 ; 0 0 0 0 0 ; 0 0 0 0 0 ;0 0 0 0 0]  Multiplication=Matrix(K*u)
  Integrator : Integrator
  Pole Pairs : Gain  Gain=MOTOR.P
  Product : Product  RndMeth=Zero
  Rr : Gain  Gain=MOTOR.Rr
  Sum : Sum  Inputs=-+
  Sum1 : Sum  Inputs=+-
  Flux r : Outport  VectorParamsAs1DForOutWhenUnconnected=off
  wires:
  Sum/1 -> Product/2
  Pole Pairs/1 -> Sum/1
  wm/1 -> Pole Pairs/1
  Gain1/1 -> Product/1
  Integrator/1 -> Gain1/1, Flux r/1
  Sum1/1 -> Integrator/1
  wframe/1 -> Sum/2
  Rr/1 -> Sum1/2
  Product/1 -> Sum1/1
  Ir_abxyz/1 -> Rr/1

== system ELECTRIC_DRIVE/MOTOR/Variant Subsystem/IM_6Ph/Stator Flux  ==
  Is_abxyz : Inport
  Vs_abxyz : Inport  Port=2
  wframe : Inport  Port=3
  Gain : Gain  Gain=[0 1 0 0 0 0;-1 0 0 0 0 0;0 0 0 0 0 0;0 0 0 0 0 0;0 0 0 0 0 0;0 0 0 0 0 0]  Multiplication=Matrix(K*u)
  Integrator : Integrator
  Product : Product  RndMeth=Zero
  Rs : Gain  Gain=MOTOR.Rs
  Sum : Sum  Inputs=+-+
  Flux s : Outport  VectorParamsAs1DForOutWhenUnconnected=off
  wires:
  Gain/1 -> Product/2
  wframe/1 -> Product/1
  Product/1 -> Sum/3
  Vs_abxyz/1 -> Sum/1
  Is_abxyz/1 -> Rs/1
  Integrator/1 -> Flux s/1, Gain/1
  Sum/1 -> Integrator/1
  Rs/1 -> Sum/2

== system ELECTRIC_DRIVE/MOTOR/Variant Subsystem/IM_6Ph/Transformation abxyz to phase ==
  Is_abxyz : Inport
  Ir_abxyz : Inport  Port=2
  Gain : Gain  Gain=MOTOR.invClarke  Multiplication=Matrix(K*u)
  Gain1 : Gain  Gain=MOTOR.invClarke  Multiplication=Matrix(K*u)
  Is_phase : Outport  VectorParamsAs1DForOutWhenUnconnected=off
  Ir_phase : Outport  Port=2  VectorParamsAs1DForOutWhenUnconnected=off
  wires:
  Gain1/1 -> Ir_phase/1
  Ir_abxyz/1 -> Gain1/1
  Gain/1 -> Is_phase/1
  Is_abxyz/1 -> Gain/1

== system ELECTRIC_DRIVE/MOTOR/Variant Subsystem/IM_6Ph/Transformation phase to abxyz ==
  Vs_phase : Inport
  Transformation alpha-beta-x-y-z : Gain  Gain=MOTOR.Clarke  Multiplication=Matrix(K*u)
  Vs_abxyz : Outport  VectorParamsAs1DForOutWhenUnconnected=off
  wires:
  Vs_phase/1 -> Transformation alpha-beta-x-y-z/1
  Transformation alpha-beta-x-y-z/1 -> Vs_abxyz/1

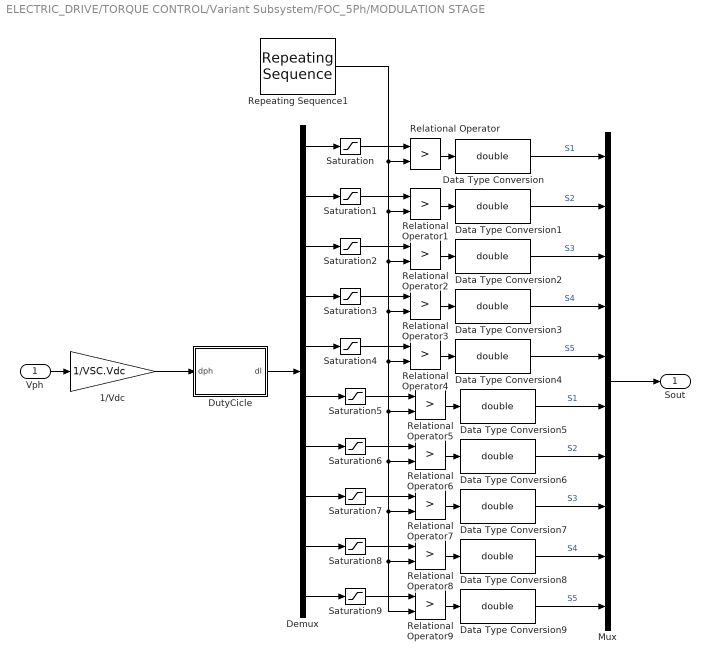
== system ELECTRIC_DRIVE/TORQUE CONTROL/Variant Subsystem/FOC_5Ph/MODULATION STAGE ==
  Vph : Inport
  1/Vdc : Gain  Gain=1/VSC.Vdc
  Data Type Conversion{,1..9} (10 alike) : DataTypeConversion  OutDataTypeStr=double  SaturateOnIntegerOverflow=off  RndMeth=Floor
  Demux : Demux  Outputs=10
  DutyCicle : MATLAB Function  TreatAsAtomicUnit=on
  Mux : Mux  Inputs=10
  Relational Operator{,1..9} (10 alike) : RelationalOperator  Operator=>  OutDataTypeStr=boolean  RndMeth=Simplest  InputSameDT=off
  Repeating Sequence1 : simulink/Sources/Repeating Sequence  rep_seq_t="[CONTROL.Tm        CONTROL.Ts/2+CONTROL.Tm        CONTROL.Ts+CONTROL.Tm ]"  rep_seq_y=[0 1 0]
  Saturation{,1..9} (10 alike) : Saturate  UpperLimit=1  LowerLimit=0
  Sout : Outport
  wires:
  Saturation1/1 -> Relational Operator1/1
  Data Type Conversion/1 -> Mux/1  "S1"
  Saturation2/1 -> Relational Operator2/1
  Data Type Conversion2/1 -> Mux/3  "S3"
  Relational Operator1/1 -> Data Type Conversion1/1
  Relational Operator2/1 -> Data Type Conversion2/1
  Saturation/1 -> Relational Operator/1
  Vph/1 -> 1/Vdc/1
  Demux/1 -> Saturation/1
  Demux/3 -> Saturation2/1
  Mux/1 -> Sout/1
  Demux/2 -> Saturation1/1
  Relational Operator/1 -> Data Type Conversion/1
  Data Type Conversion1/1 -> Mux/2  "S2"
  Data Type Conversion3/1 -> Mux/4  "S4"
  Relational Operator4/1 -> Data Type Conversion4/1
  Relational Operator3/1 -> Data Type Conversion3/1
  Data Type Conversion4/1 -> Mux/5  "S5"
  Saturation4/1 -> Relational Operator4/1
  Saturation3/1 -> Relational Operator3/1
  Demux/4 -> Saturation3/1
  Demux/5 -> Saturation4/1
  1/Vdc/1 -> DutyCicle/1(dph)
  DutyCicle/1(dl) -> Demux/1
  Demux/10 -> Saturation9/1
  Demux/9 -> Saturation8/1
  Saturation8/1 -> Relational Operator8/1
  Saturation9/1 -> Relational Operator9/1
  Data Type Conversion9/1 -> Mux/10  "S5"
  Relational Operator8/1 -> Data Type Conversion8/1
  Relational Operator9/1 -> Data Type Conversion9/1
  Repeating Sequence1/1 -> Relational Operator5/2, Relational Operator6/2, Relational Operator7/2, Relational Operator8/2, Relational Operator9/2, Relational Operator4/2, Relational Operator3/2, Relational Operator2/2, Relational Operator1/2, Relational Operator/2
  Data Type Conversion8/1 -> Mux/9  "S4"
  Data Type Conversion6/1 -> Mux/7  "S2"
  Relational Operator5/1 -> Data Type Conversion5/1
  Demux/7 -> Saturation6/1
  Demux/8 -> Saturation7/1
  Demux/6 -> Saturation5/1
  Saturation5/1 -> Relational Operator5/1
  Relational Operator7/1 -> Data Type Conversion7/1
  Relational Operator6/1 -> Data Type Conversion6/1
  Data Type Conversion7/1 -> Mux/8  "S3"
  Saturation7/1 -> Relational Operator7/1
  Data Type Conversion5/1 -> Mux/6  "S1"
  Saturation6/1 -> Relational Operator6/1

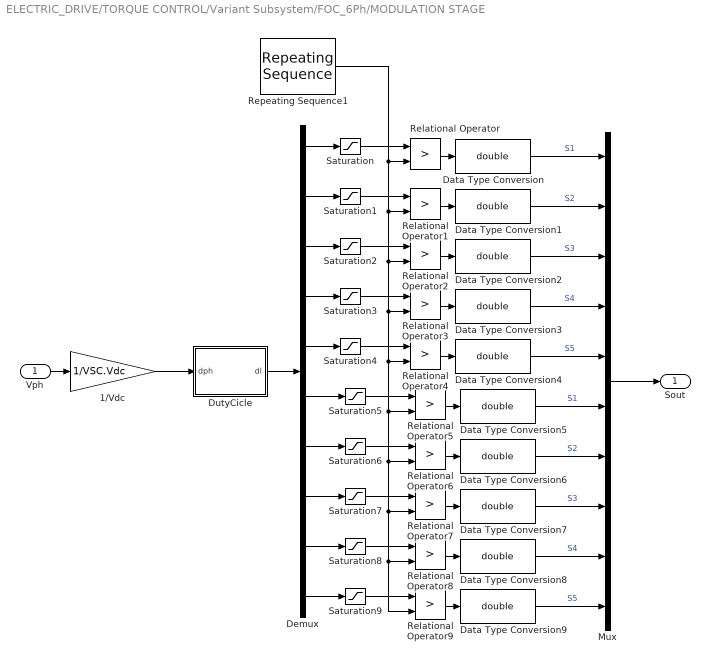
== system ELECTRIC_DRIVE/TORQUE CONTROL/Variant Subsystem/FOC_6Ph/MODULATION STAGE ==
  Vph : Inport
  1/Vdc : Gain  Gain=1/VSC.Vdc
  Data Type Conversion{,1..9} (10 alike) : DataTypeConversion  OutDataTypeStr=double  SaturateOnIntegerOverflow=off  RndMeth=Floor
  Demux : Demux  Outputs=10
  DutyCicle : MATLAB Function  TreatAsAtomicUnit=on
  Mux : Mux  Inputs=10
  Relational Operator{,1..9} (10 alike) : RelationalOperator  Operator=>  OutDataTypeStr=boolean  RndMeth=Simplest  InputSameDT=off
  Repeating Sequence1 : simulink/Sources/Repeating Sequence  rep_seq_t="[CONTROL.Tm        CONTROL.Ts/2+CONTROL.Tm        CONTROL.Ts+CONTROL.Tm ]"  rep_seq_y=[0 1 0]
  Saturation{,1..9} (10 alike) : Saturate  UpperLimit=1  LowerLimit=0
  Sout : Outport
  wires:
  Saturation6/1 -> Relational Operator6/1
  Data Type Conversion5/1 -> Mux/6  "S1"
  Saturation7/1 -> Relational Operator7/1
  Data Type Conversion7/1 -> Mux/8  "S3"
  Relational Operator6/1 -> Data Type Conversion6/1
  Relational Operator7/1 -> Data Type Conversion7/1
  Saturation5/1 -> Relational Operator5/1
  Demux/6 -> Saturation5/1
  Demux/8 -> Saturation7/1
  Demux/7 -> Saturation6/1
  Relational Operator5/1 -> Data Type Conversion5/1
  Data Type Conversion6/1 -> Mux/7  "S2"
  Data Type Conversion8/1 -> Mux/9  "S4"
  Repeating Sequence1/1 -> Relational Operator/2, Relational Operator1/2, Relational Operator2/2, Relational Operator3/2, Relational Operator4/2, Relational Operator9/2, Relational Operator8/2, Relational Operator7/2, Relational Operator6/2, Relational Operator5/2
  Relational Operator9/1 -> Data Type Conversion9/1
  Relational Operator8/1 -> Data Type Conversion8/1
  Data Type Conversion9/1 -> Mux/10  "S5"
  Saturation9/1 -> Relational Operator9/1
  Saturation8/1 -> Relational Operator8/1
  Demux/9 -> Saturation8/1
  Demux/10 -> Saturation9/1
  DutyCicle/1(dl) -> Demux/1
  1/Vdc/1 -> DutyCicle/1(dph)
  Demux/5 -> Saturation4/1
  Demux/4 -> Saturation3/1
  Saturation3/1 -> Relational Operator3/1
  Saturation4/1 -> Relational Operator4/1
  Data Type Conversion4/1 -> Mux/5  "S5"
  Relational Operator3/1 -> Data Type Conversion3/1
  Relational Operator4/1 -> Data Type Conversion4/1
  Data Type Conversion3/1 -> Mux/4  "S4"
  Data Type Conversion1/1 -> Mux/2  "S2"
  Relational Operator/1 -> Data Type Conversion/1
  Demux/2 -> Saturation1/1
  Mux/1 -> Sout/1
  Demux/3 -> Saturation2/1
  Demux/1 -> Saturation/1
  Vph/1 -> 1/Vdc/1
  Saturation/1 -> Relational Operator/1
  Relational Operator2/1 -> Data Type Conversion2/1
  Relational Operator1/1 -> Data Type Conversion1/1
  Data Type Conversion2/1 -> Mux/3  "S3"
  Saturation2/1 -> Relational Operator2/1
  Data Type Conversion/1 -> Mux/1  "S1"
  Saturation1/1 -> Relational Operator1/1

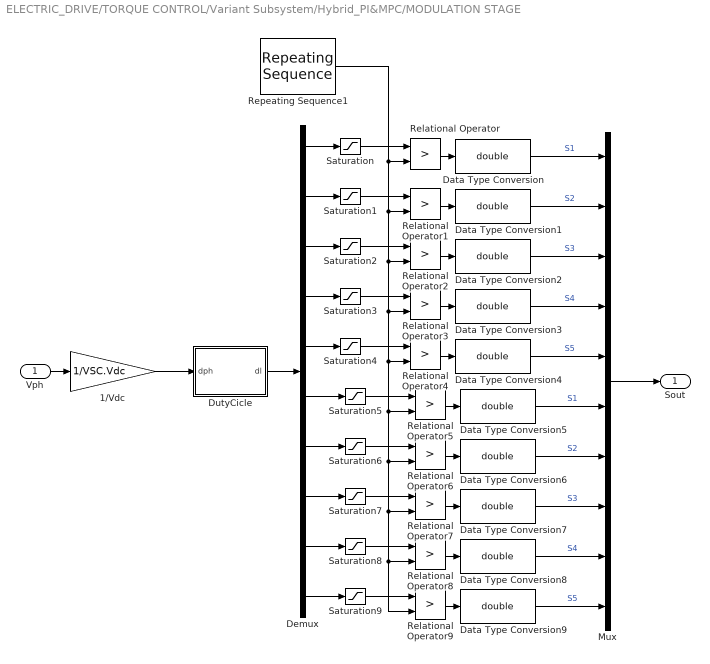
== system ELECTRIC_DRIVE/TORQUE CONTROL/Variant Subsystem/Hybrid_PI&MPC/MODULATION STAGE ==
  Vph : Inport
  1/Vdc : Gain  Gain=1/VSC.Vdc
  Data Type Conversion{,1..9} (10 alike) : DataTypeConversion  OutDataTypeStr=double  SaturateOnIntegerOverflow=off  RndMeth=Floor
  Demux : Demux  Outputs=10
  DutyCicle : MATLAB Function  TreatAsAtomicUnit=on
  Mux : Mux  Inputs=10
  Relational Operator{,1..9} (10 alike) : RelationalOperator  Operator=>  OutDataTypeStr=boolean  RndMeth=Simplest  InputSameDT=off
  Repeating Sequence1 : simulink/Sources/Repeating Sequence  rep_seq_t="[CONTROL.Tm        CONTROL.Ts/2+CONTROL.Tm        CONTROL.Ts+CONTROL.Tm ]"  rep_seq_y=[0 1 0]
  Saturation{,1..9} (10 alike) : Saturate  UpperLimit=1  LowerLimit=0
  Sout : Outport
  wires:
  Saturation6/1 -> Relational Operator6/1
  Data Type Conversion5/1 -> Mux/6  "S1"
  Saturation7/1 -> Relational Operator7/1
  Data Type Conversion7/1 -> Mux/8  "S3"
  Relational Operator6/1 -> Data Type Conversion6/1
  Relational Operator7/1 -> Data Type Conversion7/1
  Saturation5/1 -> Relational Operator5/1
  Demux/6 -> Saturation5/1
  Demux/8 -> Saturation7/1
  Demux/7 -> Saturation6/1
  Relational Operator5/1 -> Data Type Conversion5/1
  Data Type Conversion6/1 -> Mux/7  "S2"
  Data Type Conversion8/1 -> Mux/9  "S4"
  Repeating Sequence1/1 -> Relational Operator/2, Relational Operator1/2, Relational Operator2/2, Relational Operator3/2, Relational Operator4/2, Relational Operator9/2, Relational Operator8/2, Relational Operator7/2, Relational Operator6/2, Relational Operator5/2
  Relational Operator9/1 -> Data Type Conversion9/1
  Relational Operator8/1 -> Data Type Conversion8/1
  Data Type Conversion9/1 -> Mux/10  "S5"
  Saturation9/1 -> Relational Operator9/1
  Saturation8/1 -> Relational Operator8/1
  Demux/9 -> Saturation8/1
  Demux/10 -> Saturation9/1
  DutyCicle/1(dl) -> Demux/1
  1/Vdc/1 -> DutyCicle/1(dph)
  Demux/5 -> Saturation4/1
  Demux/4 -> Saturation3/1
  Saturation3/1 -> Relational Operator3/1
  Saturation4/1 -> Relational Operator4/1
  Data Type Conversion4/1 -> Mux/5  "S5"
  Relational Operator3/1 -> Data Type Conversion3/1
  Relational Operator4/1 -> Data Type Conversion4/1
  Data Type Conversion3/1 -> Mux/4  "S4"
  Data Type Conversion1/1 -> Mux/2  "S2"
  Relational Operator/1 -> Data Type Conversion/1
  Demux/2 -> Saturation1/1
  Mux/1 -> Sout/1
  Demux/3 -> Saturation2/1
  Demux/1 -> Saturation/1
  Vph/1 -> 1/Vdc/1
  Saturation/1 -> Relational Operator/1
  Relational Operator2/1 -> Data Type Conversion2/1
  Relational Operator1/1 -> Data Type Conversion1/1
  Data Type Conversion2/1 -> Mux/3  "S3"
  Saturation2/1 -> Relational Operator2/1
  Data Type Conversion/1 -> Mux/1  "S1"
  Saturation1/1 -> Relational Operator1/1

== system ELECTRIC_DRIVE/TORQUE CONTROL/Variant Subsystem/Vf_5Ph/MODULATOR ==
  Vphase : Inport
  1/Vdc : Gain  Gain=1/VSC.Vdc
  Data Type Conversion{,1..4} (5 alike) : DataTypeConversion  OutDataTypeStr=double  SaturateOnIntegerOverflow=off  RndMeth=Floor
  Demux : Demux  Outputs=5
  Mux : Mux  Inputs=5
  Relational Operator{,1..4} (5 alike) : RelationalOperator  Operator=>  OutDataTypeStr=boolean  RndMeth=Simplest  InputSameDT=off
  Repeating Sequence1 : simulink/Sources/Repeating Sequence  rep_seq_t=[0 CONTROL.Ts/2 CONTROL.Ts ]  rep_seq_y=[-1 1 -1]/2
  Scope : Scope  NumInputPorts=2
  Sout : Outport
  wires:
  Relational Operator1/1 -> Data Type Conversion1/1
  Relational Operator4/1 -> Data Type Conversion4/1
  Relational Operator3/1 -> Data Type Conversion3/1
  Data Type Conversion3/1 -> Mux/4
  Relational Operator2/1 -> Data Type Conversion2/1
  Demux/5 -> Relational Operator4/1
  Demux/2 -> Relational Operator1/1
  Demux/3 -> Relational Operator2/1
  Mux/1 -> Sout/1
  Repeating Sequence1/1 -> Scope/1, Relational Operator4/2, Relational Operator3/2, Relational Operator2/2, Relational Operator1/2, Relational Operator/2
  Data Type Conversion2/1 -> Mux/3  "Sc"
  Demux/1 -> Scope/2, Relational Operator/1
  Relational Operator/1 -> Data Type Conversion/1
  Data Type Conversion/1 -> Mux/1  "Sa"
  Data Type Conversion4/1 -> Mux/5
  Demux/4 -> Relational Operator3/1
  Vphase/1 -> 1/Vdc/1
  1/Vdc/1 -> Demux/1
  Data Type Conversion1/1 -> Mux/2  "Sb"

== system ELECTRIC_DRIVE/MOTOR/Variant Subsystem/IM_5Ph/Current/falta ==
  I_alpha : Inport
  Ix : Inport  Port=2
  Clock : Clock
  Gain1 : Gain  Gain=-1
  Switch : Switch  Criteria=u2 > Threshold  Threshold=tfalta  SaturateOnIntegerOverflow=off  InputSameDT=off
  Ix1 : Outport  VectorParamsAs1DForOutWhenUnconnected=off
  wires:
  Ix/1 -> Switch/3
  Switch/1 -> Ix1/1
  Clock/1 -> Switch/2
  I_alpha/1 -> Gain1/1
  Gain1/1 -> Switch/1

== matlab function ELECTRIC_DRIVE/MOTOR/Variant Subsystem/PMSM_5Ph/ab2dq1 ==
  data: Iabxy input; Idqxy output; th input
 function Idqxy = Park(Iabxy,th)

% Mp= [ cos(th)   sin(th)           0         0          0
%      -sin(th)   cos(th)           0         0          0 
%          0           0        cos(3*th)   -sin(3*th)   0
%          0           0        sin(3*th)    cos(3*th)   0
%          0           0            0         0          1];
Idqxy = zeros(5,1);
Mp= [ cos(th)   sin(th)  0  0  0
     -sin(th)   cos(th)  0  0  0 
         0           0    cos(3*th)   sin(3*th)  0
         0           0   -sin(3*th)   cos(3*th)  0
         0           0   0  0  1];

Idqxy = Mp*Iabxy;
end

== matlab function ELECTRIC_DRIVE/MOTOR/Variant Subsystem/IM_5Ph/ab2dq ==
  data: Vabxy input; Vdqxy output; th input
 function Vdqxy = Park(Vabxy,th)

% Mp= [ cos(th)   sin(th)           0         0          0
%      -sin(th)   cos(th)           0         0          0 
%          0           0        cos(3*th)   -sin(3*th)   0
%          0           0        sin(3*th)    cos(3*th)   0
%          0           0            0         0          1];
Vdqxy = zeros(5,1);
Mp= [ cos(th)   sin(th)  0  0  
     -sin(th)   cos(th)  0  0  
         0           0   1  0  
         0           0   0  1 ];

Vdqxy = Mp*Vabxy;
end

== matlab function ELECTRIC_DRIVE/TORQUE CONTROL/Variant Subsystem/MPC_5Ph_PMSM/MPC 5Phase PMSM ==
  settings: updateMethod=DISCRETE
  data: Iabc_med input; Sout output; Tref input; wm input; th input; CONTROL parameter; SENSOR parameter; vectores output; Fc_out output; IdqRef output; IabRef output; Iab_km1 output; ch output
function [Sout, vectores, Fc_out, IdqRef, IabRef, Iab_km1, ch] = FCS_MPC_5PH_PMSM(Iabc_med, Tref, wm, th, CONTROL, SENSOR)

% Variable init
persistent uk;
persistent cntr;
persistent x_opt;
% persistent Fc_ana;
persistent Fc;
persistent J_opt;
persistent dq_ref;
persistent Iab_ref;
persistent Sout_km1;
persistent cambios;
persistent Iabxy_med;
persistent xkp1;
persistent Pkm1;

persistent th_km2;

persistent GAMMA;
persistent GAMMA_Vab;

if isempty(cntr)
    uk  = [0 0 0 0 0]';
    cntr= CONTROL.N_calc;
    Iab_ref = zeros(5,1);
    xkp1 = zeros(5,1);
    dq_ref = zeros(5,1);
    % Fc_ana = zeros(3*length(V_abxy) ,1);
    Fc     = 0;
    Sout_km1 = zeros(length(CONTROL.VECT.S(:,1)),1);
    Sout = zeros(length(CONTROL.VECT.S(:,1)),1);
    cambios = 0;
    x_opt = 0;
    Iabxy_med = zeros(CONTROL.Phase,1);

    Pkm1 = zeros(5,5);

    th_km2 = th;

    GAMMA = CONTROL.B * CONTROL.Ts;
    GAMMA_Vab = GAMMA * CONTROL.Vdc*CONTROL.VECT.V_abxy;
end


%---------  CONTROL LOOP  ---------%
if (cntr==CONTROL.N_calc)
    cntr=0;

    we=wm*CONTROL.P;               % Electric speed
    th_km2 = th + 2*CONTROL.Ts*we; % Orientation correction

    %----- REFERENCE CURRENTS -----%
    Id_ref  = 0;
    Iq_ref  = (2/CONTROL.Phase) * Tref/(CONTROL.P*CONTROL.Lambda); 
    Id2_ref = 0;
    Iq2_ref = 0;
    Ih_ref  = 0;

    % Saturation
    if (Iq_ref >= CONTROL.In)
        Iq_ref = CONTROL.In;
    elseif (Iq_ref <= -CONTROL.In)
        Iq_ref = -CONTROL.In;
    end

    % Inverse Park transform
    Ia_ref = Id_ref*cos(th_km2)    - Iq_ref*sin(th_km2);
    Ib_ref = Id_ref*sin(th_km2)    + Iq_ref*cos(th_km2);
    Ix_ref = Id2_ref*cos(3*th_km2) - Iq2_ref*sin(3*th_km2);
    Iy_ref = Id2_ref*sin(3*th_km2) + Iq2_ref*cos(3*th_km2);

    dq_ref  = [Id_ref Iq_ref Id2_ref Iq2_ref Ih_ref]';
    Iab_ref = [Ia_ref Ib_ref Ix_ref  Iy_ref  Ih_ref]';

    %-----   STATE SPACE   -----%
    Ap=[ 0    -((CONTROL.Ld-CONTROL.Lq)*we)/CONTROL.Ld 0  0  0
    ((CONTROL.Ld-CONTROL.Lq)*we)/CONTROL.Lq  0         0  0  0
         0                                   0         0  0  0
         0                                   0         0  0  0
         0                                   0         0  0  0];
    FI=(eye(CONTROL.Phase) + (CONTROL.A+Ap) *CONTROL.Ts); % Discrete state space

    Bemf = we* CONTROL.E.* [sin(th)   % A-B X-Y frame
                            cos(th)
                            sin(3*th)
                            cos(3*th)
                            sin(5*th)];

    %-----  CURRENT MEASUREMENT  -----%
    Iph_sensor = Iabc_med + SENSOR.CURRENT.sigma*randn(5,1);
    
    %  Filtro de Kalman 
    if CONTROL.KALMAN.ACTIVE == 1
        Iph_k = CONTROL.invClarke * xkp1;
        Pk = FI*Pkm1*inv(FI) + CONTROL.KALMAN.Q;
        kk = Pk*inv(Pk + CONTROL.KALMAN.R);
        
        Iph_filt = Iph_k + kk*(Iph_sensor - Iph_k);
        Pkm1 = (eye(5)-kk)*Pk;
    else
        Iph_filt = Iph_sensor;
    end

    Iabxy_med = CONTROL.Clarke*Iph_filt;
    xk = [Iabxy_med(1) Iabxy_med(2) Iabxy_med(3) Iabxy_med(4) Iabxy_med(5)]';

    %----- PREDICTION k+1 -----%
    xkp1=FI*xk + GAMMA*(uk + Bemf);

    %----- PREDICTION k+2 (CONSTANT) -----%
    xkp2_cnst = FI*xkp1 + Bemf*CONTROL.Ts;

    %---- OPTIMIZATION LOOP - PREDICTION k+2 ----%
    J_opt = inf; %Inicializacion de la funcion de coste
    for m=1:length(CONTROL.VECT.indx)
        xkp2  = xkp2_cnst + GAMMA_Vab(:,CONTROL.VECT.indx(m));% xkp2  = FI*xkp1 + GAMMA*V_abxy(:,m) + DELTA;
        error = Iab_ref - xkp2;

        Fc1 = error(1)^2 + CONTROL.Kd*error(2)^2;
        Fc2 = CONTROL.Kx*error(3)^2 + CONTROL.Ky*error(4)^2;
        Fc3 = CONTROL.Kh*(error(5)^2);    % Fc_ana(m) = Fc1; Fc_ana(m + length(V_abxy)) = Fc2; Fc_ana(m + 2*length(V_abxy)) = Fc3;

        Fc = Fc1 + Fc2 + Fc3;

        if (Fc < J_opt)
            J_opt=Fc;
            x_opt = m;
        end
    end
    % Voltage vector update
    uk = CONTROL.Vdc*CONTROL.VECT.V_abxy(:,CONTROL.VECT.indx(x_opt));

    % Swith_km2ing frec. calculation
    cambios = cambios + sum(abs(CONTROL.VECT.S(:,CONTROL.VECT.indx(x_opt)) - Sout_km1)); 
    Sout_km1 = CONTROL.VECT.S(:,CONTROL.VECT.indx(x_opt));
end
cntr = cntr + 1;

%----- ACTUATION -----%
Sout = Sout_km1;

% Output Variable Update
IdqRef = dq_ref;
IabRef = Iab_ref;
Iab_km1 = xkp1;
Fc_out = Fc;
vectores = CONTROL.VECT.indx(x_opt);
ch = cambios;
end
